simulink model "tester"  (R2024a)
settings: Solver=VariableStepAuto  StartTime=0.0  StopTime=inf  RelTol=1e-3
undefined symbols (not defined in the file): dt, I_charge_max, I_max, Id_char, Imax, Ion, Iq_char, Ki_d, Ki_q, Kp_d, Kp_q, lambda, Ld, Lithium, Lq, p, Rs, Soc_max, V_batt, Vdc_nom, Vs_max
libraries: mcbcontrolslib x4, simulink x2, spsBatteryLib x1, spsPermanentMagnetSynchronousMachineLib x1, spsSeriesRLCBranchLib x1, spsThreePhaseFaultLib x1, spsUniversalBridgeLib x1, sps_lib x1
(part 2 of 2)

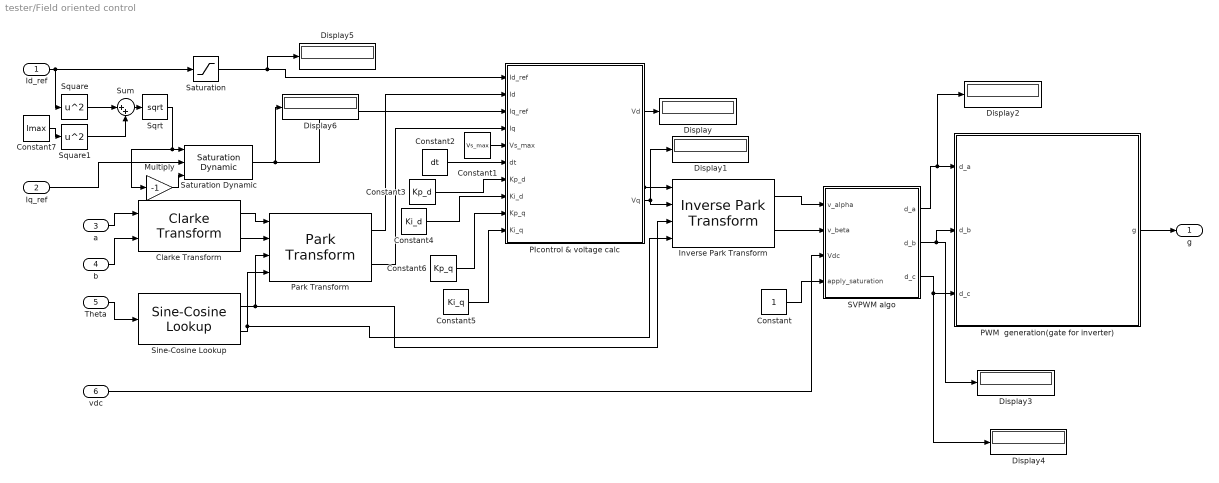
== system tester/Field oriented control ==
  Id_ref : Inport
  Iq_ref : Inport  Port=2
  a : Inport  Port=3
  b : Inport  Port=4
  Theta : Inport  Port=5
  vdc : Inport  Port=6
  Clarke Transform : mcbcontrolslib/Clarke Transform  VariantControl=Variant2  PhaseInput=Two inputs  EnPowerInv=off
      settings: LibrarySourceBlock=mcbhdllib/Controls/Math Transforms/Clarke Transform
  Constant : Constant
  Constant1 : Constant  Value=Vs_max
  Constant2 : Constant  Value=dt
  Constant3 : Constant  Value=Kp_d
  Constant4 : Constant  Value=Ki_d
  Constant5 : Constant  Value=Ki_q
  Constant6 : Constant  Value=Kp_q
  Constant7 : Constant  Value=Imax
  Display{,1..6} (7 alike) : Display
  Inverse Park Transform : mcbcontrolslib/Inverse Park Transform  PhaseInput=Two inputs  AxisAlignment=D-axis  ThetaInput=Sine and Cosine electrical position  AngleInput=Per-unit  N_points=1024
      settings: LibrarySourceBlock=mcbhdllib/Controls/Math Transforms/Inverse Park Transform
  Multiply : Gain  Gain=-1
  PIcontrol & voltage calc : MATLAB Function  TreatAsAtomicUnit=on
  PWM  generation(gate for inverter) : Subsystem
  Park Transform : mcbcontrolslib/Park Transform  PhaseInput=Two inputs  AxisAlignment=D-axis  ThetaInput=Sine and Cosine electrical position  AngleInput=Per-unit  N_points=1024
      settings: LibrarySourceBlock=mcbhdllib/Controls/Math Transforms/Park Transform
  SVPWM algo : MATLAB Function  TreatAsAtomicUnit=on
  Saturation : Saturate  UpperLimit=I_max  LowerLimit=-Imax
  Saturation Dynamic : simulink/Discontinuities/Saturation Dynamic  OutMin=[]  OutMax=[]  OutDataTypeStr=Inherit: Same as second input  OutDataType=fixdt(1, 16)  OutScaling=2^-10  DoSatur=off
  Sine-Cosine Lookup : mcbcontrolslib/Sine-Cosine Lookup  AngleInput=Per-unit  N_points=1024  DatatypeInput=Inherit from input  Datatype=single
      settings: LibrarySourceBlock=mcblib/Controls/Math Transforms/Sine-Cosine Lookup
  Sqrt : Sqrt
  Square : Math  Operator=square
  Square1 : Math  Operator=square
  Sum : Sum  Inputs=|++
  g : Outport
  wires:
  b/1 -> Clarke Transform/2
  Clarke Transform/1 -> Park Transform/1
  a/1 -> Clarke Transform/1
  Sine-Cosine Lookup/2 -> Inverse Park Transform/4, Park Transform/4
  PIcontrol & voltage calc/1(Vd) -> Display/1, Inverse Park Transform/1
  Clarke Transform/2 -> Park Transform/2
  Park Transform/1 -> PIcontrol & voltage calc/2(Id)
  Sine-Cosine Lookup/1 -> Inverse Park Transform/3, Park Transform/3
  PIcontrol & voltage calc/2(Vq) -> Inverse Park Transform/2, Display1/1
  Id_ref/1 -> Square/1, Saturation/1
  Park Transform/2 -> PIcontrol & voltage calc/4(Iq)
  Theta/1 -> Sine-Cosine Lookup/1
  Inverse Park Transform/1 -> SVPWM algo/1(v_alpha)
  Inverse Park Transform/2 -> SVPWM algo/2(v_beta)
  vdc/1 -> SVPWM algo/3(Vdc)
  Constant/1 -> SVPWM algo/4(apply_saturation)
  SVPWM algo/1(d_a) -> Display2/1, PWM  generation(gate for inverter)/1(d_a)
  SVPWM algo/2(d_b) -> Display3/1, PWM  generation(gate for inverter)/2(d_b)
  SVPWM algo/3(d_c) -> Display4/1, PWM  generation(gate for inverter)/3(d_c)
  PWM  generation(gate for inverter)/1(g) -> g/1
  Constant1/1 -> PIcontrol & voltage calc/5(Vs_max)
  Constant2/1 -> PIcontrol & voltage calc/6(dt)
  Constant3/1 -> PIcontrol & voltage calc/7(Kp_d)
  Constant4/1 -> PIcontrol & voltage calc/8(Ki_d)
  Constant5/1 -> PIcontrol & voltage calc/10(Ki_q)
  Constant6/1 -> PIcontrol & voltage calc/9(Kp_q)
  Saturation/1 -> Display5/1, PIcontrol & voltage calc/1(Id_ref)
  Square/1 -> Sum/1
  Constant7/1 -> Square1/1
  Square1/1 -> Sum/2
  Sum/1 -> Sqrt/1
  Sqrt/1 -> Multiply/1, Saturation Dynamic/1
  Iq_ref/1 -> Saturation Dynamic/2
  Multiply/1 -> Saturation Dynamic/3
  Saturation Dynamic/1 -> Display6/1, PIcontrol & voltage calc/3(Iq_ref)

== system tester/References Calculation ==
  Regen_availability : Inport
  TrqREq : Inport  Port=2
  Wm : Inport  Port=3
  Base speed calculation : Subsystem
  MTPA  torque calculation : Subsystem
  MTPA current references : Subsystem
  Mode Determination + (dq) references genration : Subsystem
  Torque reference determination : Subsystem
  Voltages Calculation : Subsystem
  Id_ref : Outport
  Iq_ref : Outport  Port=2
  wires:
  Torque reference determination/1(Tref) -> Mode Determination + (dq) references genration/1(Tref), MTPA current references/1(T_ref)
  MTPA current references/2(Iq_ref_mtpa) -> Voltages Calculation/2(Iq_ref_mtpa), Mode Determination + (dq) references genration/4(Iq_ref_mtpa)
  TrqREq/1 -> Torque reference determination/1(TrqReq)
  MTPA current references/1(Id_ref_mtpa) -> Mode Determination + (dq) references genration/2(Id_ref_mtpa), Voltages Calculation/1(Id_ref_mtpa)
  Voltages Calculation/1(Vd_mtpa) -> Mode Determination + (dq) references genration/3(Vd_mtpa)
  Wm/1 -> Torque reference determination/4(Wmech), Mode Determination + (dq) references genration/6(Wmech), Voltages Calculation/3(Wmech)
  [T_mtpa_max] -> Torque reference determination/3(T_mtpa_max)
  MTPA  torque calculation/1(T_mtpa_max) -> [T_mtpa_max]
  Voltages Calculation/2(Vq_mtpa) -> Mode Determination + (dq) references genration/5(Vq_mtpa)
  Mode Determination + (dq) references genration/2(Iq_ref) -> Iq_ref/1
  Mode Determination + (dq) references genration/1(Id_ref) -> Id_ref/1
  Regen_availability/1 -> Torque reference determination/2(Regen_availability)
  Base speed calculation/1(Wbase) -> Mode Determination + (dq) references genration/7(Wbase)

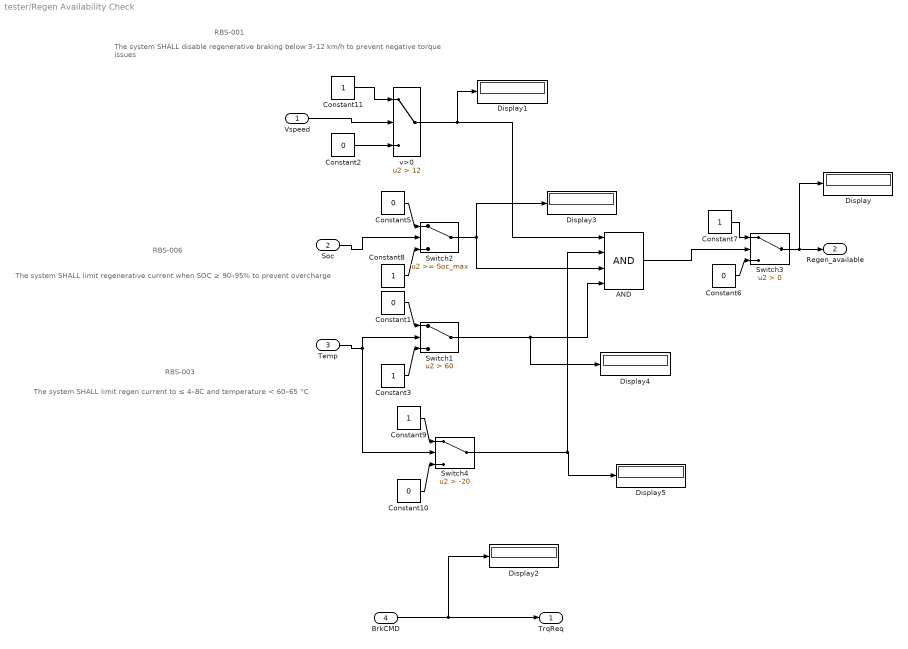
== system tester/Regen Availability Check ==
  note: RBS-006
  note: The system SHALL limit regenerative current when SOC ≥ 90–95% to prevent overcharge
  note: RBS-003
  note: The system SHALL limit regen current to ≤ 4–8C and temperature < 60–65 °C
  note: RBS-001
  note: The system SHALL disable regenerative braking below 3–12 km/h to prevent negative torque issues
  Vspeed : Inport
  Soc : Inport  Port=2
  Temp : Inport  Port=3
  BrkCMD : Inport  Port=4
  AND : Logic  Inputs=4  IconShape=distinctive  AllPortsSameDT=off  OutDataTypeStr=boolean
  Constant{1,5..6,10} (4 alike) : Constant  Value=0
  Constant{3,7..9,11} (5 alike) : Constant
  Constant2 : Constant  Value=0  SampleTime=-1
  Display{,1..5} (6 alike) : Display
  Switch1 : Switch  Criteria=u2 > Threshold  Threshold=60  SaturateOnIntegerOverflow=off  InputSameDT=off
  Switch2 : Switch  Threshold=Soc_max  SaturateOnIntegerOverflow=off  InputSameDT=off
  Switch3 : Switch  Criteria=u2 > Threshold  SaturateOnIntegerOverflow=off  InputSameDT=off
  Switch4 : Switch  Criteria=u2 > Threshold  Threshold=-20  SaturateOnIntegerOverflow=off  InputSameDT=off
  v>0 : Switch  Criteria=u2 > Threshold  Threshold=12  SaturateOnIntegerOverflow=off  InputSameDT=off
  TrqReq : Outport  VectorParamsAs1DForOutWhenUnconnected=off
  Regen_available : Outport  Port=2
  wires:
  Constant2/1 -> v>0/3
  Vspeed/1 -> v>0/2
  Constant11/1 -> v>0/1
  Constant6/1 -> Switch3/3
  Constant7/1 -> Switch3/1
  AND/1 -> Switch3/2
  Switch3/1 -> Display/1, Regen_available/1
  v>0/1 -> Display1/1, AND/1
  Soc/1 -> Switch2/2
  Constant8/1 -> Switch2/3
  Constant5/1 -> Switch2/1
  Temp/1 -> Switch4/2, Switch1/2
  Constant3/1 -> Switch1/3
  Constant1/1 -> Switch1/1
  Constant10/1 -> Switch4/3
  Constant9/1 -> Switch4/1
  Switch2/1 -> AND/3, Display3/1
  Switch1/1 -> Display4/1, AND/4
  Switch4/1 -> AND/2, Display5/1
  BrkCMD/1 -> Display2/1, TrqReq/1

== system tester/Subsystem ==
  In1 : Inport
  Display : Display
  Display1 : Display
  Multiply : Gain  Gain=250
  Multiply1 : Gain  Gain=1500
  Vspeed : Outport
  Wm : Outport  Port=2
  wires:
  Multiply/1 -> Display/1, Vspeed/1
  In1/1 -> Multiply1/1, Multiply/1
  Multiply1/1 -> Display1/1, Wm/1

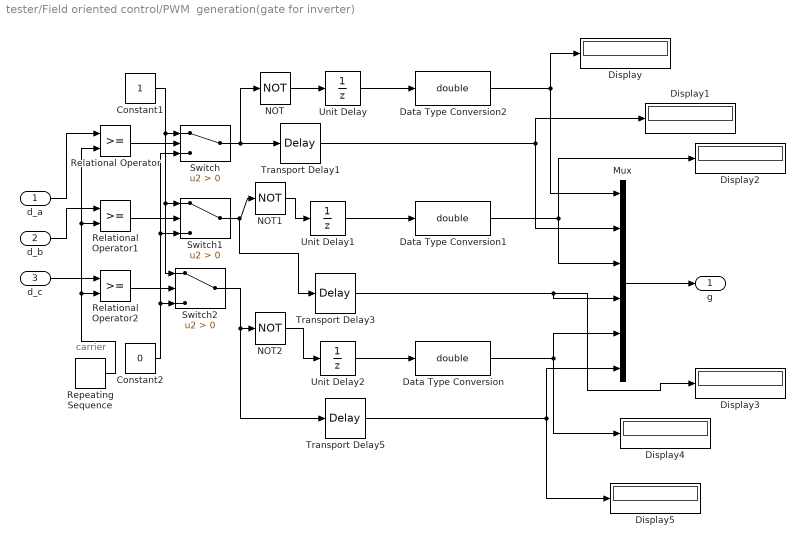
== system tester/Field oriented control/PWM  generation(gate for inverter) ==
  note: carrier
  d_a : Inport
  d_b : Inport  Port=2
  d_c : Inport  Port=3
  Constant1 : Constant
  Constant2 : Constant  Value=0
  Data Type Conversion : DataTypeConversion  OutDataTypeStr=double  SaturateOnIntegerOverflow=off  RndMeth=Floor
  Data Type Conversion1 : DataTypeConversion  OutDataTypeStr=double  SaturateOnIntegerOverflow=off  RndMeth=Floor
  Data Type Conversion2 : DataTypeConversion  OutDataTypeStr=double  SaturateOnIntegerOverflow=off  RndMeth=Floor
  Display{,1..5} (6 alike) : Display
  Mux : Mux  Inputs=6
  NOT : Logic  Operator=NOT  IconShape=distinctive  AllPortsSameDT=off  OutDataTypeStr=boolean
  NOT1 : Logic  Operator=NOT  IconShape=distinctive  AllPortsSameDT=off  OutDataTypeStr=boolean
  NOT2 : Logic  Operator=NOT  IconShape=distinctive  AllPortsSameDT=off  OutDataTypeStr=boolean
  Relational Operator : RelationalOperator  OutDataTypeStr=boolean  RndMeth=Simplest  InputSameDT=off
  Relational Operator1 : RelationalOperator  OutDataTypeStr=boolean  RndMeth=Simplest  InputSameDT=off
  Relational Operator2 : RelationalOperator  OutDataTypeStr=boolean  RndMeth=Simplest  InputSameDT=off
  Repeating Sequence : simulink/Sources/Repeating Sequence  rep_seq_t=[0, 0.5, 1]*1e-4  rep_seq_y=[0, 1, 0]
  Switch : Switch  Criteria=u2 > Threshold  SaturateOnIntegerOverflow=off  InputSameDT=off
  Switch1 : Switch  Criteria=u2 > Threshold  SaturateOnIntegerOverflow=off  InputSameDT=off
  Switch2 : Switch  Criteria=u2 > Threshold  SaturateOnIntegerOverflow=off  InputSameDT=off
  Transport Delay1 : TransportDelay  DelayTime=300e-9
  Transport Delay3 : TransportDelay  DelayTime=300e-9
  Transport Delay5 : TransportDelay  DelayTime=300e-9
  Unit Delay : UnitDelay  SampleTime=-1  HasFrameUpgradeWarning=on
  Unit Delay1 : UnitDelay  SampleTime=-1  HasFrameUpgradeWarning=on
  Unit Delay2 : UnitDelay  SampleTime=-1  HasFrameUpgradeWarning=on
  g : Outport
  wires:
  Repeating Sequence/1 -> Relational Operator2/2, Relational Operator1/2, Relational Operator/2
  NOT2/1 -> Unit Delay2/1
  Switch2/1 -> Transport Delay5/1, NOT2/1
  Unit Delay/1 -> Data Type Conversion2/1
  Constant1/1 -> Switch2/1, Switch1/1, Switch/1
  Mux/1 -> g/1
  NOT1/1 -> Unit Delay1/1
  Switch/1 -> Transport Delay1/1, NOT/1
  Constant2/1 -> Switch/3, Switch1/3, Switch2/3
  Switch1/1 -> Transport Delay3/1, NOT1/1
  Unit Delay1/1 -> Data Type Conversion1/1
  Transport Delay1/1 -> Display1/1, Mux/2
  Relational Operator/1 -> Switch/2
  d_c/1 -> Relational Operator2/1
  Transport Delay5/1 -> Mux/6, Display5/1
  Transport Delay3/1 -> Display3/1, Mux/4
  Unit Delay2/1 -> Data Type Conversion/1
  Relational Operator1/1 -> Switch1/2
  Relational Operator2/1 -> Switch2/2
  d_a/1 -> Relational Operator/1
  d_b/1 -> Relational Operator1/1
  NOT/1 -> Unit Delay/1
  Data Type Conversion2/1 -> Display/1, Mux/1
  Data Type Conversion1/1 -> Display2/1, Mux/3
  Data Type Conversion/1 -> Mux/5, Display4/1

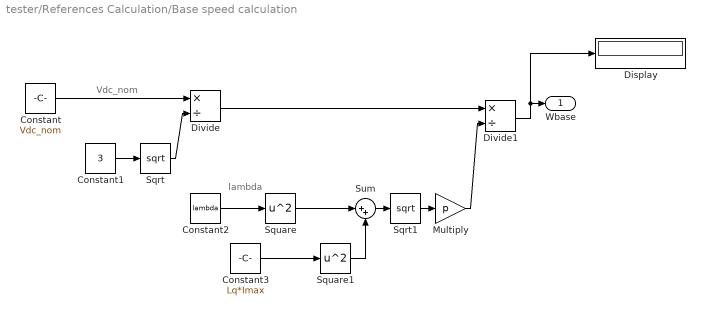
== system tester/References Calculation/Base speed calculation ==
  note: Vdc_nom
  note: lambda
  Constant : Constant  Value=Vdc_nom
  Constant1 : Constant  Value=3
  Constant2 : Constant  Value=lambda
  Constant3 : Constant  Value=Lq*Imax
  Display : Display
  Divide : Product  Inputs=*/
  Divide1 : Product  Inputs=*/
  Multiply : Gain  Gain=p
  Sqrt : Sqrt
  Sqrt1 : Sqrt
  Square : Math  Operator=square
  Square1 : Math  Operator=square
  Sum : Sum  Inputs=|++
  Wbase : Outport
  wires:
  Sqrt/1 -> Divide/2
  Constant/1 -> Divide/1
  Multiply/1 -> Divide1/2
  Divide1/1 -> Display/1, Wbase/1
  Sum/1 -> Sqrt1/1
  Constant3/1 -> Square1/1
  Constant2/1 -> Square/1
  Square1/1 -> Sum/2
  Constant1/1 -> Sqrt/1
  Divide/1 -> Divide1/1
  Sqrt1/1 -> Multiply/1
  Square/1 -> Sum/1

== system tester/References Calculation/MTPA  torque calculation ==
  Constant : Constant  Value=Imax
  Constant1 : Constant  Value=Ld
  Constant2 : Constant  Value=Lq
  Constant3 : Constant  Value=lambda
  Display : Display
  MATLAB Function : MATLAB Function  TreatAsAtomicUnit=on
  T_mtpa_max : Outport
  wires:
  Constant1/1 -> MATLAB Function/2(Ld)
  Constant3/1 -> MATLAB Function/4(lambda_pm)
  Constant/1 -> MATLAB Function/1(I_max)
  MATLAB Function/1(T_mtpa_max) -> Display/1, T_mtpa_max/1
  Constant2/1 -> MATLAB Function/3(Lq)

== system tester/References Calculation/MTPA current references ==
  T_ref : Inport
  Calculate MTPA reference currents : MATLAB Function  TreatAsAtomicUnit=on
  Constant : Constant  Value=Ld
  Constant1 : Constant  Value=Lq
  Constant2 : Constant  Value=lambda
  Constant3 : Constant  Value=p
  Constant4 : Constant  Value=I_max
  Display : Display
  Display1 : Display
  Id_ref_mtpa : Outport
  Iq_ref_mtpa : Outport  Port=2
  wires:
  Calculate MTPA reference currents/2(Iq_ref) -> Display1/1, Iq_ref_mtpa/1
  Constant1/1 -> Calculate MTPA reference currents/3(Lq)
  Calculate MTPA reference currents/1(Id_ref) -> Display/1, Id_ref_mtpa/1
  Constant/1 -> Calculate MTPA reference currents/2(Ld)
  T_ref/1 -> Calculate MTPA reference currents/1(T_ref)
  Constant2/1 -> Calculate MTPA reference currents/4(lambda_pm)
  Constant3/1 -> Calculate MTPA reference currents/5(p)
  Constant4/1 -> Calculate MTPA reference currents/6(I_max)

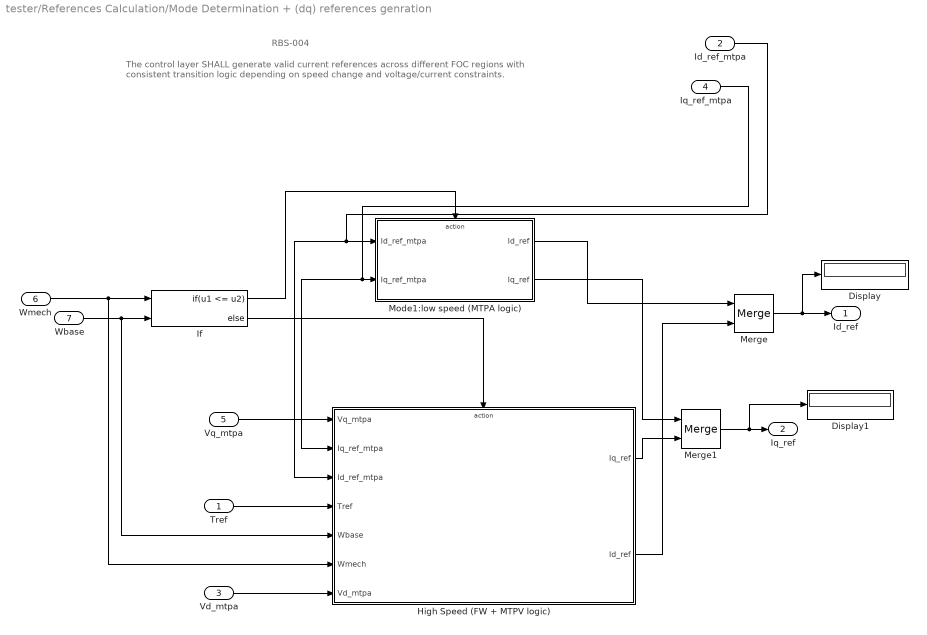
== system tester/References Calculation/Mode Determination + (dq) references genration ==
  note: RBS-004
  note: The control layer SHALL generate valid current references across different FOC regions with consistent transition logic depending on speed change and voltage/current constraints.
  Tref : Inport
  Id_ref_mtpa : Inport  Port=2
  Vd_mtpa : Inport  Port=3
  Iq_ref_mtpa : Inport  Port=4
  Vq_mtpa : Inport  Port=5
  Wmech : Inport  Port=6
  Wbase : Inport  Port=7
  Display : Display
  Display1 : Display
  High Speed (FW + MTPV logic) : Subsystem  TreatAsAtomicUnit=on
  If : If  NumInputs=2  IfExpression=u1 <= u2
  Merge : Merge
  Merge1 : Merge
  Mode1:low speed (MTPA logic) : Subsystem  TreatAsAtomicUnit=on
  Id_ref : Outport
  Iq_ref : Outport  Port=2
  wires:
  Wmech/1 -> High Speed (FW + MTPV logic)/6(Wmech), If/1
  If/2 -> High Speed (FW + MTPV logic)/Action
  Wbase/1 -> High Speed (FW + MTPV logic)/5(Wbase), If/2
  Mode1:low speed (MTPA logic)/1(Id_ref) -> Merge/1
  Mode1:low speed (MTPA logic)/2(Iq_ref) -> Merge1/1
  High Speed (FW + MTPV logic)/1(Iq_ref) -> Merge1/2
  Iq_ref_mtpa/1 -> High Speed (FW + MTPV logic)/2(Iq_ref_mtpa), Mode1:low speed (MTPA logic)/2(Iq_ref_mtpa)
  If/1 -> Mode1:low speed (MTPA logic)/Action
  Id_ref_mtpa/1 -> High Speed (FW + MTPV logic)/3(Id_ref_mtpa), Mode1:low speed (MTPA logic)/1(Id_ref_mtpa)
  Vd_mtpa/1 -> High Speed (FW + MTPV logic)/7(Vd_mtpa)
  Vq_mtpa/1 -> High Speed (FW + MTPV logic)/1(Vq_mtpa)
  Tref/1 -> High Speed (FW + MTPV logic)/4(Tref)
  Merge1/1 -> Display1/1, Iq_ref/1
  Merge/1 -> Display/1, Id_ref/1
  High Speed (FW + MTPV logic)/2(Id_ref) -> Merge/2

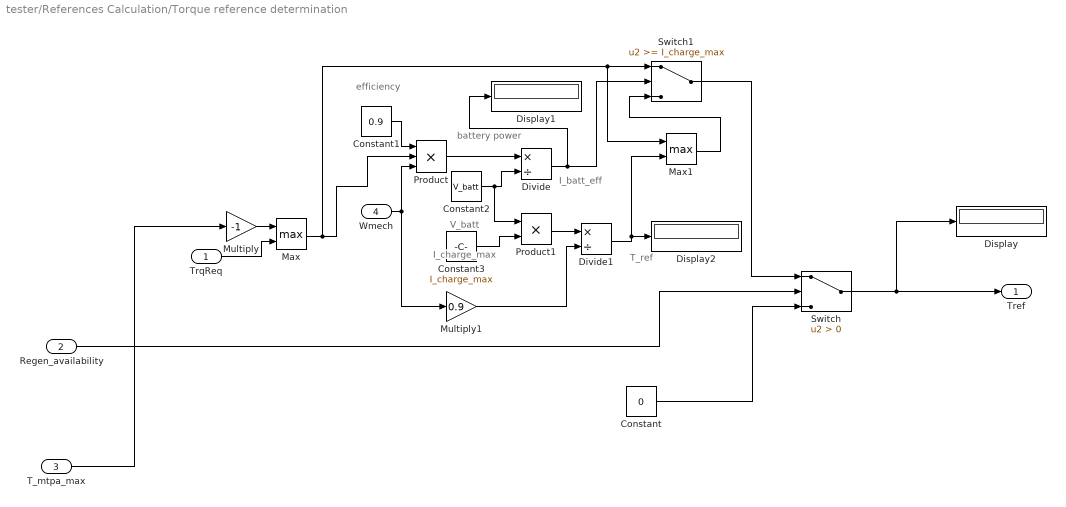
== system tester/References Calculation/Torque reference determination ==
  note: T_ref
  note: I_batt_eff
  note: V_batt
  note: I_charge_max
  note: battery power
  note: efficiency
  TrqReq : Inport
  Regen_availability : Inport  Port=2
  T_mtpa_max : Inport  Port=3
  Wmech : Inport  Port=4
  Constant : Constant  Value=0
  Constant1 : Constant  Value=0.9
  Constant2 : Constant  Value=V_batt
  Constant3 : Constant  Value=I_charge_max
  Display : Display
  Display1 : Display
  Display2 : Display
  Divide : Product  Inputs=*/
  Divide1 : Product  Inputs=*/
  Max : MinMax  Function=max  Inputs=2
  Max1 : MinMax  Function=max  Inputs=2
  Multiply : Gain  Gain=-1
  Multiply1 : Gain  Gain=0.9
  Product : Product  Inputs=3
  Product1 : Product
  Switch : Switch  Criteria=u2 > Threshold  SaturateOnIntegerOverflow=off  InputSameDT=off
  Switch1 : Switch  Threshold=I_charge_max  SaturateOnIntegerOverflow=off  InputSameDT=off
  Tref : Outport
  wires:
  Divide1/1 -> Max1/2, Display2/1
  Multiply1/1 -> Divide1/2
  Max/1 -> Max1/1, Switch1/1, Product/2
  Wmech/1 -> Multiply1/1, Product/3
  Multiply/1 -> Max/1
  Constant2/1 -> Product1/1, Divide/2
  Product/1 -> Divide/1
  Constant1/1 -> Product/1
  Product1/1 -> Divide1/1
  Constant3/1 -> Product1/2
  Divide/1 -> Display1/1, Switch1/2
  Constant/1 -> Switch/3
  Switch1/1 -> Switch/1
  TrqReq/1 -> Max/2
  T_mtpa_max/1 -> Multiply/1
  Regen_availability/1 -> Switch/2
  Switch/1 -> Display/1, Tref/1
  Max1/1 -> Switch1/3

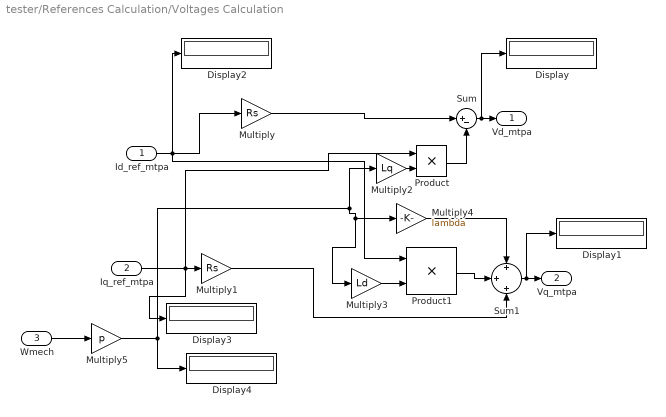
== system tester/References Calculation/Voltages Calculation ==
  Id_ref_mtpa : Inport
  Iq_ref_mtpa : Inport  Port=2
  Wmech : Inport  Port=3
  Display{,1..4} (5 alike) : Display
  Multiply : Gain  Gain=Rs
  Multiply1 : Gain  Gain=Rs
  Multiply2 : Gain  Gain=Lq
  Multiply3 : Gain  Gain=Ld
  Multiply4 : Gain  Gain=lambda
  Multiply5 : Gain  Gain=p
  Product : Product
  Product1 : Product
  Sum : Sum  Inputs=|+-
  Sum1 : Sum  Inputs=+|+|+
  Vd_mtpa : Outport
  Vq_mtpa : Outport  Port=2
  wires:
  Iq_ref_mtpa/1 -> Display3/1, Product/1, Multiply1/1
  Id_ref_mtpa/1 -> Display2/1, Product1/1, Multiply/1
  Product/1 -> Sum/2
  Multiply/1 -> Sum/1
  Multiply5/1 -> Multiply4/1, Multiply3/1, Multiply2/1, Display4/1
  Multiply2/1 -> Product/2
  Multiply4/1 -> Sum1/1
  Sum/1 -> Display/1, Vd_mtpa/1
  Multiply3/1 -> Product1/2
  Product1/1 -> Sum1/2
  Multiply1/1 -> Sum1/3
  Sum1/1 -> Display1/1, Vq_mtpa/1
  Wmech/1 -> Multiply5/1

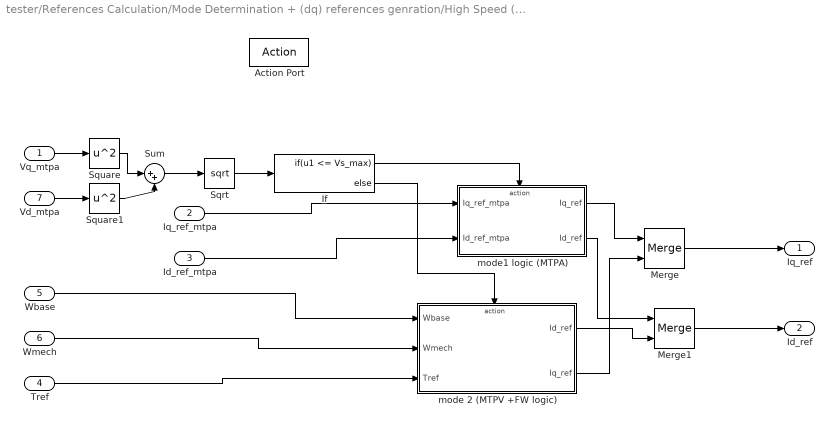
== system tester/References Calculation/Mode Determination + (dq) references genration/High Speed (FW + MTPV logic) ==
  Vq_mtpa : Inport
  Iq_ref_mtpa : Inport  Port=2
  Id_ref_mtpa : Inport  Port=3
  Tref : Inport  Port=4
  Wbase : Inport  Port=5
  Wmech : Inport  Port=6
  Vd_mtpa : Inport  Port=7
  Action Port : ActionPort  ActionPortLabel=else
  If : If  IfExpression=u1 <= Vs_max
  Merge : Merge
  Merge1 : Merge
  Sqrt : Sqrt
  Square : Math  Operator=square
  Square1 : Math  Operator=square
  Sum : Sum  Inputs=|++
  mode 2 (MTPV +FW logic) : Subsystem  TreatAsAtomicUnit=on
  mode1 logic (MTPA) : Subsystem  TreatAsAtomicUnit=on
  Iq_ref : Outport
  Id_ref : Outport  Port=2
  wires:
  Vq_mtpa/1 -> Square/1
  Vd_mtpa/1 -> Square1/1
  Square/1 -> Sum/1
  Square1/1 -> Sum/2
  Sum/1 -> Sqrt/1
  Sqrt/1 -> If/1
  If/1 -> mode1 logic (MTPA)/Action
  Iq_ref_mtpa/1 -> mode1 logic (MTPA)/1(Iq_ref_mtpa)
  Id_ref_mtpa/1 -> mode1 logic (MTPA)/2(Id_ref_mtpa)
  If/2 -> mode 2 (MTPV +FW logic)/Action
  Wbase/1 -> mode 2 (MTPV +FW logic)/1(Wbase)
  Wmech/1 -> mode 2 (MTPV +FW logic)/2(Wmech)
  Tref/1 -> mode 2 (MTPV +FW logic)/3(Tref)
  mode1 logic (MTPA)/1(Iq_ref) -> Merge/1
  mode 2 (MTPV +FW logic)/2(Iq_ref) -> Merge/2
  mode1 logic (MTPA)/2(Id_ref) -> Merge1/1
  mode 2 (MTPV +FW logic)/1(Id_ref) -> Merge1/2
  Merge/1 -> Iq_ref/1
  Merge1/1 -> Id_ref/1

== system tester/References Calculation/Mode Determination + (dq) references genration/Mode1:low speed (MTPA logic) ==
  Id_ref_mtpa : Inport
  Iq_ref_mtpa : Inport  Port=2
  Action Port : ActionPort  ActionPortLabel=if(u1 <= u2)
  Constant : Constant  Value=I_max
  Display : Display
  Display1 : Display
  mode1:low speed(MTPA refrences) : MATLAB Function  TreatAsAtomicUnit=on
  Id_ref : Outport
  Iq_ref : Outport  Port=2
  wires:
  Id_ref_mtpa/1 -> mode1:low speed(MTPA refrences)/1(Id_ref_mtpa)
  Iq_ref_mtpa/1 -> mode1:low speed(MTPA refrences)/2(Iq_ref_mtpa)
  mode1:low speed(MTPA refrences)/1(Id_ref) -> Display/1, Id_ref/1
  mode1:low speed(MTPA refrences)/2(Iq_ref) -> Display1/1, Iq_ref/1
  Constant/1 -> mode1:low speed(MTPA refrences)/3(I_max)

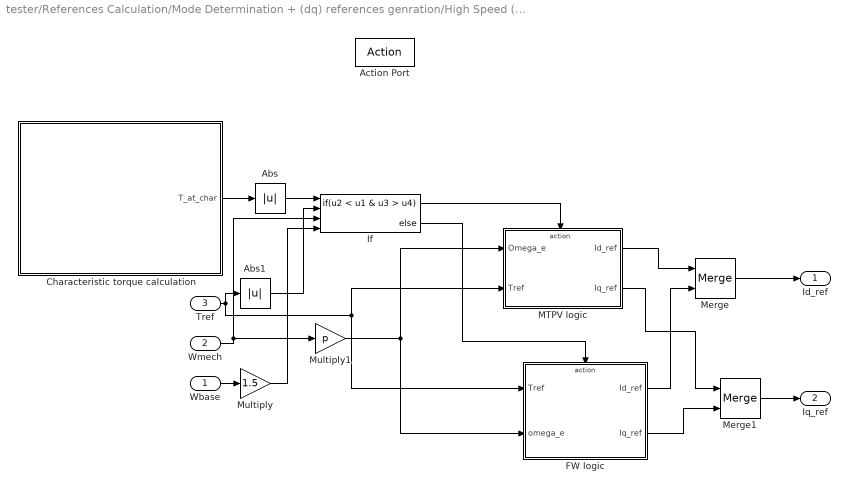
== system tester/References Calculation/Mode Determination + (dq) references genration/High Speed (FW + MTPV logic)/mode 2 (MTPV +FW logic) ==
  Wbase : Inport
  Wmech : Inport  Port=2
  Tref : Inport  Port=3
  Action Port : ActionPort  ActionPortLabel=else
  Abs : Abs  SaturateOnIntegerOverflow=off
  Abs1 : Abs  SaturateOnIntegerOverflow=off
  Characteristic torque calculation : Subsystem
  FW logic : Subsystem  TreatAsAtomicUnit=on
  If : If  NumInputs=4  IfExpression=u2 < u1 & u3 > u4
  MTPV logic : Subsystem  TreatAsAtomicUnit=on
  Merge : Merge
  Merge1 : Merge
  Multiply : Gain  Gain=1.5
  Multiply1 : Gain  Gain=p
  Id_ref : Outport
  Iq_ref : Outport  Port=2
  wires:
  Characteristic torque calculation/1(T_at_char) -> Abs/1
  Abs/1 -> If/1
  Wbase/1 -> Multiply/1
  Tref/1 -> Abs1/1, FW logic/1(Tref), MTPV logic/2(Tref)
  Abs1/1 -> If/2
  Wmech/1 -> Multiply1/1, If/3
  Multiply/1 -> If/4
  If/1 -> MTPV logic/Action
  Multiply1/1 -> FW logic/2(omega_e), MTPV logic/1(Omega_e)
  If/2 -> FW logic/Action
  FW logic/1(Id_ref) -> Merge/2
  MTPV logic/1(Id_ref) -> Merge/1
  FW logic/2(Iq_ref) -> Merge1/2
  MTPV logic/2(Iq_ref) -> Merge1/1
  Merge/1 -> Id_ref/1
  Merge1/1 -> Iq_ref/1

== system tester/References Calculation/Mode Determination + (dq) references genration/High Speed (FW + MTPV logic)/mode1 logic (MTPA) ==
  Iq_ref_mtpa : Inport
  Id_ref_mtpa : Inport  Port=2
  Action Port : ActionPort  ActionPortLabel=if(u1 <= Vs_max)
  Iq_ref : Outport
  Id_ref : Outport  Port=2
  wires:
  Iq_ref_mtpa/1 -> Iq_ref/1
  Id_ref_mtpa/1 -> Id_ref/1

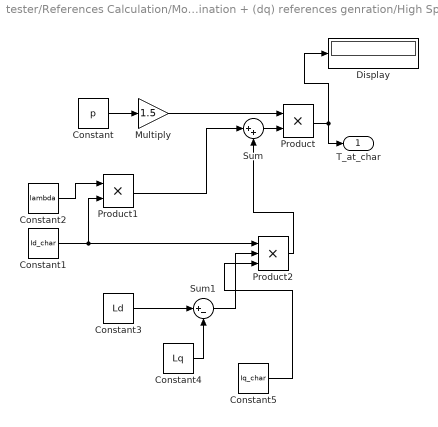
== system tester/References Calculation/Mode Determination + (dq) references genration/High Speed (FW + MTPV logic)/mode 2 (MTPV +FW logic)/Characteristic torque calculation ==
  Constant : Constant  Value=p
  Constant1 : Constant  Value=Id_char
  Constant2 : Constant  Value=lambda
  Constant3 : Constant  Value=Ld
  Constant4 : Constant  Value=Lq
  Constant5 : Constant  Value=Iq_char
  Display : Display
  Multiply : Gain  Gain=1.5
  Product : Product
  Product1 : Product
  Product2 : Product  Inputs=3
  Sum : Sum  Inputs=|++
  Sum1 : Sum  Inputs=|+-
  T_at_char : Outport
  wires:
  Product1/1 -> Sum/1
  Product/1 -> Display/1, T_at_char/1
  Sum1/1 -> Product2/2
  Constant3/1 -> Sum1/1
  Constant2/1 -> Product1/1
  Sum/1 -> Product/2
  Product2/1 -> Sum/2
  Constant4/1 -> Sum1/2
  Constant1/1 -> Product2/1, Product1/2
  Constant/1 -> Multiply/1
  Multiply/1 -> Product/1
  Constant5/1 -> Product2/3

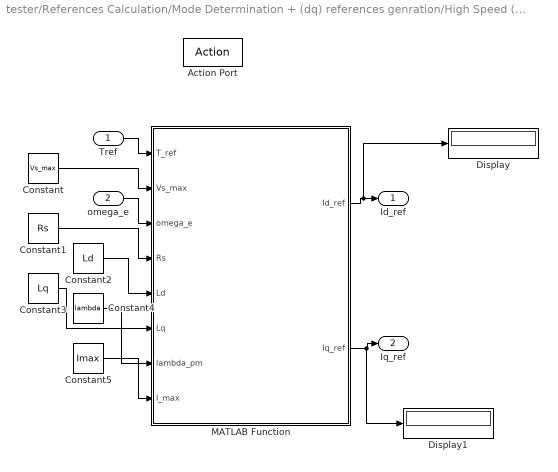
== system tester/References Calculation/Mode Determination + (dq) references genration/High Speed (FW + MTPV logic)/mode 2 (MTPV +FW logic)/FW logic ==
  Tref : Inport
  omega_e : Inport  Port=2
  Action Port : ActionPort  ActionPortLabel=else
  Constant : Constant  Value=Vs_max
  Constant1 : Constant  Value=Rs
  Constant2 : Constant  Value=Ld
  Constant3 : Constant  Value=Lq
  Constant4 : Constant  Value=lambda
  Constant5 : Constant  Value=Imax
  Display : Display
  Display1 : Display
  MATLAB Function : MATLAB Function  TreatAsAtomicUnit=on
  Id_ref : Outport
  Iq_ref : Outport  Port=2
  wires:
  Tref/1 -> MATLAB Function/1(T_ref)
  omega_e/1 -> MATLAB Function/3(omega_e)
  Constant/1 -> MATLAB Function/2(Vs_max)
  Constant1/1 -> MATLAB Function/4(Rs)
  Constant2/1 -> MATLAB Function/5(Ld)
  Constant3/1 -> MATLAB Function/6(Lq)
  Constant4/1 -> MATLAB Function/7(lambda_pm)
  Constant5/1 -> MATLAB Function/8(I_max)
  MATLAB Function/1(Id_ref) -> Display/1, Id_ref/1
  MATLAB Function/2(Iq_ref) -> Display1/1, Iq_ref/1

== system tester/References Calculation/Mode Determination + (dq) references genration/High Speed (FW + MTPV logic)/mode 2 (MTPV +FW logic)/MTPV logic ==
  Omega_e : Inport
  Tref : Inport  Port=2
  Action Port : ActionPort  ActionPortLabel=if(u2 < u1 & u3 > u4)
  Constant : Constant  Value=Vs_max
  Constant1 : Constant  Value=Rs
  Constant2 : Constant  Value=Ld
  Constant3 : Constant  Value=Lq
  Constant4 : Constant  Value=lambda
  Constant5 : Constant  Value=I_max
  Display : Display
  Display1 : Display
  MATLAB Function : MATLAB Function  TreatAsAtomicUnit=on
  Id_ref : Outport
  Iq_ref : Outport  Port=2
  wires:
  Omega_e/1 -> MATLAB Function/3(omega_e)
  Tref/1 -> MATLAB Function/1(T_ref)
  Constant/1 -> MATLAB Function/2(Vs_max)
  Constant1/1 -> MATLAB Function/4(Rs)
  Constant2/1 -> MATLAB Function/5(Ld)
  Constant3/1 -> MATLAB Function/6(Lq)
  Constant4/1 -> MATLAB Function/7(lambda_pm)
  MATLAB Function/1(Id_ref) -> Display/1, Id_ref/1
  MATLAB Function/2(Iq_ref) -> Display1/1, Iq_ref/1
  Constant5/1 -> MATLAB Function/8(I_max)

== matlab function tester/Field oriented control/SVPWM algo ==
  data: v_alpha input; d_a output; v_beta input; Vdc input; apply_saturation input; d_b output; d_c output
function [d_a, d_b, d_c] = svpwm_step(v_alpha, v_beta, Vdc, apply_saturation)
% SVPWM_STEP - Space Vector PWM duty cycle generation
%
% Inputs:
%   v_alpha          : Alpha-axis voltage reference [V]
%   v_beta           : Beta-axis voltage reference [V]
%   Vdc              : DC bus voltage [V]
%   apply_saturation : 1 = scale vector to linear region, 0 = skip
%
% Outputs:
%   d_a    : Phase A duty cycle [0 to 1]
%   d_b    : Phase B duty cycle [0 to 1]
%   d_c    : Phase C duty cycle [0 to 1]
%   overmod: Overmodulation flag (1 = exceeded linear region)
%   scale  : Scaling factor applied (1.0 = no scaling)

    %% Input protection
    if Vdc <= 0
        %error('Vdc must be greater than 0');
    end

    %% Step 1 — Voltage Saturation (optional)
    v_lim = Vdc / sqrt(3);
    mag   = sqrt(v_alpha^2 + v_beta^2);

    if apply_saturation && mag > v_lim && mag > 1e-12
        scale       = v_lim / mag;
        v_alpha_use = v_alpha * scale;
        v_beta_use  = v_beta  * scale;
    else
        scale       = 1.0;
        v_alpha_use = v_alpha;
        v_beta_use  = v_beta;
    end

    %% Step 2 — Alpha-Beta to ABC (line-neutral references)
    v_a =  v_alpha_use;
    v_b = -0.5 * v_alpha_use + (sqrt(3)/2) * v_beta_use;
    v_c = -0.5 * v_alpha_use - (sqrt(3)/2) * v_beta_use;

    %% Step 3 — Zero-sequence injection (SVPWM offset)
    v_max = max([v_a, v_b, v_c]);
    v_min = min([v_a, v_b, v_c]);
    v_0   = -0.5 * (v_max + v_min);

    v_a0 = v_a + v_0;
    v_b0 = v_b + v_0;
    v_c0 = v_c + v_0;

    %% Step 4 — Duty cycle mapping
    d_a_raw = 0.5 + (v_a0 / Vdc);
    d_b_raw = 0.5 + (v_b0 / Vdc);
    d_c_raw = 0.5 + (v_c0 / Vdc);

    %% Step 6 — Clamp duties to [0, 1]
    d_a = min(max(d_a_raw, 0), 1);
    d_b = min(max(d_b_raw, 0), 1);
    d_c = min(max(d_c_raw, 0), 1);

end

== matlab function tester/References Calculation/MTPA  torque calculation/MATLAB Function ==
  data: I_max input; T_mtpa_max output; Ld input; Lq input; lambda_pm input
function T_mtpa_max = calculate_mtpa_torque(I_max, Ld, Lq, lambda_pm)
    % Calculate maximum torque under MTPA with current limit
    % For IPMSM: T = 1.5*p*(λ_pm*Iq + (Ld-Lq)*Id*Iq)
    % MTPA condition: Id = -(λ_pm/(2*(Ld-Lq))) - sqrt((λ_pm/(2*(Ld-Lq)))^2 + Iq^2)
    
    Iq_range = linspace(0, I_max, 1000);
    T_range = zeros(size(Iq_range));
    Id_range = zeros(size(Iq_range));
    
    for j = 1:length(Iq_range)
        Iq_j = Iq_range(j);
        % MTPA Id for given Iq
        Id_j =  (lambda_pm/(2*(Ld-Lq))) - sqrt((lambda_pm/(2*(Ld-Lq)))^2 + (Iq_j^2));
        % Check current limit
        if sqrt(Id_j^2 + Iq_j^2) <= I_max
            T_range(j) = 1.5 * (lambda_pm * Iq_j + (Ld - Lq) * Id_j * Iq_j);
            Id_range(j) = Id_j;
        end
    end
    
    [T_mtpa_max, idx] = max(T_range);
    %Id_opt = Id_range(idx);
    %Iq_opt = Iq_range(idx); %for current inspection and scope
end

== matlab function tester/References Calculation/Mode Determination + (dq) references genration/High Speed (FW + MTPV logic)/mode 2 (MTPV +FW logic)/MTPV logic/MATLAB Function ==
  data: T_ref input; Id_ref output; Vs_max input; omega_e input; Rs input; Ld input; Lq input; lambda_pm input; Iq_ref output; I_max input
function [Id_ref, Iq_ref] = calculate_mptv_currents(T_ref, Vs_max, omega_e, Rs, Ld, Lq, lambda_pm,I_max)
    % Maximum Torque Per Voltage - voltage limited operation
    
    delta_L = Ld - Lq;
    T_norm = T_ref / 1.5;
    
    % MPTV occurs at the intersection of constant torque curve and voltage ellipse
    % with maximum Id (most negative) for that torque
    
    % Start from characteristic current
    Id_char = -lambda_pm / Lq;
    Id_guess = Id_char;
    Iq_guess = T_norm / (lambda_pm + delta_L * Id_char);
    
    for iter = 1:100
        % Voltage
        Vd = Rs*Id_guess - omega_e*Lq*Iq_guess;
        Vq = Rs*Iq_guess + omega_e*Ld*Id_guess + omega_e*lambda_pm;
        Vs = sqrt(Vd^2 + Vq^2);
        
        % Torque
        T_calc = lambda_pm * Iq_guess + delta_L * Id_guess * Iq_guess;
        
        err_V = Vs - Vs_max;
        err_T = T_calc - T_norm;
        
        % Adjust
        dId = 0.5;
        Vd_plus = Rs*(Id_guess+dId) - omega_e*Lq*Iq_guess;
        Vq_plus = Rs*Iq_guess + omega_e*Ld*(Id_guess+dId) + omega_e*lambda_pm;
        Vs_plus = sqrt(Vd_plus^2 + Vq_plus^2);
        dVs_dId = (Vs_plus - Vs) / dId;
        
        if abs(dVs_dId) > 1e-10
            Id_guess = Id_guess - err_V / dVs_dId;
        end
        
        if abs(lambda_pm + delta_L * Id_guess) > 1e-10
            Iq_guess = T_norm / (lambda_pm + delta_L * Id_guess);
        end
        
        if abs(err_V) < 0.1 && abs(err_T) < 0.01
            break;
        end
    end
    Id_ref = Id_guess;
    Iq_ref = Iq_guess;
end

== matlab function tester/References Calculation/Mode Determination + (dq) references genration/Mode1:low speed (MTPA logic)/mode1:low speed(MTPA refrences) ==
  data: Id_ref_mtpa input; Iq_ref_mtpa input; Id_ref output; Iq_ref output; I_max input
function [Id_ref, Iq_ref] = get_mtpa_vals(Id_ref_mtpa,Iq_ref_mtpa,I_max)
    Is_ref = sqrt(Id_ref_mtpa^2 + Iq_ref_mtpa^2);
    if Is_ref > I_max
        Id_ref_mtpa = Id_ref_mtpa * I_max / Is_ref; %assure the references are always within the limits (limitation)
        Iq_ref_mtpa = Iq_ref_mtpa * I_max / Is_ref;
    end
    Id_ref = Id_ref_mtpa;
    Iq_ref = Iq_ref_mtpa;
end

== matlab function tester/References Calculation/Mode Determination + (dq) references genration/High Speed (FW + MTPV logic)/mode 2 (MTPV +FW logic)/FW logic/MATLAB Function ==
  data: T_ref input; Id_ref output; Vs_max input; omega_e input; Rs input; Ld input; Lq input; lambda_pm input; I_max input; Iq_ref output
function [Id_ref, Iq_ref] =calculate_fw_currents(T_ref, Vs_max, omega_e, Rs, Ld, Lq, lambda_pm, I_max)
    % Field Weakening with current limit intersection
    
    delta_L = Ld - Lq;
    T_norm = T_ref / 1.5;
    
    % Iterate to find Id, Iq that satisfy both torque and voltage equations
    Id_guess = 0;
    Iq_guess = T_norm / lambda_pm;
    
    for iter = 1:100
        % Voltage equations
        Vd = Rs*Id_guess - omega_e*Lq*Iq_guess;
        Vq = Rs*Iq_guess + omega_e*Ld*Id_guess + omega_e*lambda_pm;
        Vs = sqrt(Vd^2 + Vq^2);
        
        % Torque
        T_calc = lambda_pm * Iq_guess + delta_L * Id_guess * Iq_guess;
        
        % Errors
        err_V = Vs - Vs_max;
        err_T = T_calc - T_norm;
        
        % Adjust Id (more negative = more FW)
        dId = -0.5;
        Vd_plus = Rs*(Id_guess+dId) - omega_e*Lq*Iq_guess;
        Vq_plus = Rs*Iq_guess + omega_e*Ld*(Id_guess+dId) + omega_e*lambda_pm;
        Vs_plus = sqrt(Vd_plus^2 + Vq_plus^2);
        dVs_dId = (Vs_plus - Vs) / dId;
        
        if abs(dVs_dId) > 1e-10
            Id_guess = Id_guess - err_V / dVs_dId;
        end
        
        % Adjust Iq to maintain torque
        if abs(delta_L * Id_guess) > 1e-10
            Iq_guess = T_norm / (lambda_pm + delta_L * Id_guess);
        else
            Iq_guess = T_norm / lambda_pm;
        end
        
        % Apply current limit
        Is = sqrt(Id_guess^2 + Iq_guess^2);
        if Is > I_max
            scale = I_max / Is;
            Id_guess = Id_guess * scale;
            Iq_guess = Iq_guess * scale;
        end
        
        if abs(err_V) < 0.1 && abs(err_T) < 0.01
            break;
        end
    end
    Id_ref = Id_guess;
    Iq_ref = Iq_guess;
end

== matlab function tester/References Calculation/MTPA current references/Calculate MTPA reference currents ==
  data: T_ref input; Id_ref output; Ld input; Lq input; lambda_pm input; Iq_ref output; p input; I_max input; feasible output
function [Id_ref, Iq_ref, feasible] = calculate_mtpa_currents(T_ref, Ld, Lq, lambda_pm, p, I_max)
%#codegen
% "True MTPA" by minimizing Is^2 = Id^2 + Iq^2 subject to torque equation.
% Adds current-limit feasibility check and avoids Iq near zero singularity.

    if nargin < 5 || isempty(p),     p = 3;      end
    if nargin < 6 || isempty(I_max), I_max = 580; end

    Id_ref = 0; Iq_ref = 0; feasible = true;

    if abs(T_ref) < 1e-3
        return;
    end

    Tn = T_ref / (1.5*p);     % normalized torque
    dL = (Ld - Lq);

    % Non-salient: Id=0
    if abs(dL) < 1e-12
        Iq = Tn / lambda_pm;
        if abs(Iq) > I_max
            feasible = false;
            Iq = sign(Iq)*I_max;
        end
        Id_ref = 0;
        Iq_ref = Iq;
        return;
    end

    % Scan Iq in a bounded region. For regen, Iq negative; for motoring, positive.
    Iq_max = I_max;
    N = 2001;

    if T_ref > 0
        Iq_lo =  0.02*I_max;   % avoid near-zero
        Iq_hi =  Iq_max;
    else
        Iq_lo = -Iq_max;
        Iq_hi = -0.02*I_max;   % avoid near-zero
    end

    bestJ = Inf;
    bestId = 0; bestIq = 0;
    found = false;

    for k = 0:(N-1)
        Iq = Iq_lo + (Iq_hi - Iq_lo) * (k/(N-1));

        % Torque constraint => Id
        Id = (Tn - lambda_pm*Iq) / (dL*Iq);

        Is2 = Id*Id + Iq*Iq;

        % Enforce current limit as constraint
        if Is2 <= (I_max*I_max)
            if Is2 < bestJ
                bestJ = Is2;
                bestId = Id;
                bestIq = Iq;
                found = true;
            end
        end
    end

    if ~found
        % Not feasible within I_max: fall back to saturating along Iq axis (safe/simple)
        feasible = false;
        Id_ref = 0;
        Iq_ref = sign(T_ref) * min(abs(Tn/lambda_pm), I_max);
    else
        Id_ref = bestId;
        Iq_ref = bestIq;
    end
end

== matlab function tester/Field oriented control/PIcontrol & voltage calc ==
  settings: updateMethod=DISCRETE
  data: Vd output; Id_ref input; Id input; Iq_ref input; Iq input; Vq output; Vs_max input; dt input; Kp_d input; Ki_d input; Kp_q input; Ki_q input
function [Vd, Vq] = Current_PI_control_VoltageCalc(Id_ref, Id, Iq_ref, Iq, Vs_max, dt, Kp_d, Ki_d, Kp_q, Ki_q)
%#codegen
% PI current controller with simple anti-windup and voltage magnitude limiting.
%
% Inputs:
%   Id_ref, Id, Iq_ref, Iq : currents [A]
%   Vs_max                 : max voltage magnitude (phase/space vector limit) [V]
%   dt                     : sample time [s]
%   Kp_d, Ki_d, Kp_q, Ki_q : PI gains
%
% Outputs:
%   Vd, Vq                 : dq voltage commands [V]

% Ensure scalar outputs for size inference
Vd = 0.0;
Vq = 0.0;

% Persistent integrator states
persistent int_err_Id int_err_Iq
if isempty(int_err_Id)
    int_err_Id = 0.0;
end
if isempty(int_err_Iq)
    int_err_Iq = 0.0;
end

% Anti-windup limits (axis-wise)
Vd_max = Vs_max;
Vq_max = Vs_max;

%% d-axis
err_Id = Id_ref - Id;

% integrate
int_err_Id = int_err_Id + err_Id * dt;

% PI
Vd_cmd = Kp_d * err_Id + Ki_d * int_err_Id;

% anti-windup (revert integration if saturated)
if abs(Vd_cmd) > Vd_max
    int_err_Id = int_err_Id - err_Id * dt;
    Vd_cmd = sign(Vd_cmd) * Vd_max;
end

%% q-axis
err_Iq = Iq_ref - Iq;

% integrate
int_err_Iq = int_err_Iq + err_Iq * dt;

% PI
Vq_cmd = Kp_q * err_Iq + Ki_q * int_err_Iq;

% anti-windup (revert integration if saturated)
if abs(Vq_cmd) > Vq_max
    int_err_Iq = int_err_Iq - err_Iq * dt;
    Vq_cmd = sign(Vq_cmd) * Vq_max;
end

%% Voltage limiting (vector magnitude / circle constraint)
Vs_cmd = sqrt(Vd_cmd*Vd_cmd + Vq_cmd*Vq_cmd);
if Vs_cmd > Vs_max && Vs_cmd > 1e-12
    scale = Vs_max / Vs_cmd;
    Vd_cmd = Vd_cmd * scale;
    Vq_cmd = Vq_cmd * scale;
end

Vd = Vd_cmd;
Vq = Vq_cmd;
end
